simulink model "PIME_FxNLMS_2023a"  (R2023a)
settings: Solver=VariableStepAuto  StartTime=0.0  StopTime=60  FixedStep=1/fs  RelTol=1e-3
values from neighbouring files (symbols this model uses):
  alpha = 0.999    [pime_init.m]
  c2 = 0.12    [pime_init.m]
  fs = 2000    [pime_init.m]
  k = 0.06    [pime_init.m]
  Mp = 500    [pime_init.m]
  Ms = 500    [pime_init.m]
  mu = 0.4    [pime_init.m]
  mu2 = 0.1    [pime_init.m]
  pp_mic4 = [-0.00152613187005 0.000492531757844 -0.000591319109315 0.000123902983694 0.000500734431321 -0.00102276849056 0.00131789801081 -0.000708342152862 0.00106442677388 -0.0010811148944 0.00122345086739 -0.00108254398921 ... (2000 elements, 2000x1)]    [paths_2kHz_mic643.mat]
  pp_mic6 = [0.00546659867813 -0.00630560555543 0.00626955740335 -0.00617656797871 0.00600172736047 -0.00577131330306 0.00631697277776 -0.0055608004128 0.00521354039728 -0.00486275779688 0.00518931562889 -0.00454952673028 ... (2000 elements, 2000x1)]    [paths_2kHz_mic643.mat]
  sp_mic4 = [0.0248657891061 -0.0218126639931 0.0255846134288 -0.0178527223693 0.0231404239645 0.863574751981 -0.0887369954303 -0.473837577644 -0.356836562663 -0.384364342858 -0.167933167392 -0.0752079364537 ... (2000 elements, 2000x1)]    [paths_2kHz_mic643.mat]
  sp_mic6 = [0.0393906263967 -0.0418257652999 0.0388004904193 -0.0450848758925 0.464349566334 1.5072784377 -0.746160308217 -0.827489248229 -0.750534401853 -0.550302899738 -0.217506295103 -0.0688944606907 ... (2000 elements, 2000x1)]    [paths_2kHz_mic643.mat]
  t_mic_change = 30    [pime_init.m]
undefined symbols (not defined in the file or in its folder): pp_micro6, sp_micro6
libraries: simulink x3, dspadpt3 x2, dspswit3 x2, dspsrcs4 x1, dspvision x1
settings Model: Creator=JUAGA26J  LastModifiedBy=enrole
settings DataIOCC: SaveFormat=Array
settings RTWCC: GPUComputeCapability=5.0

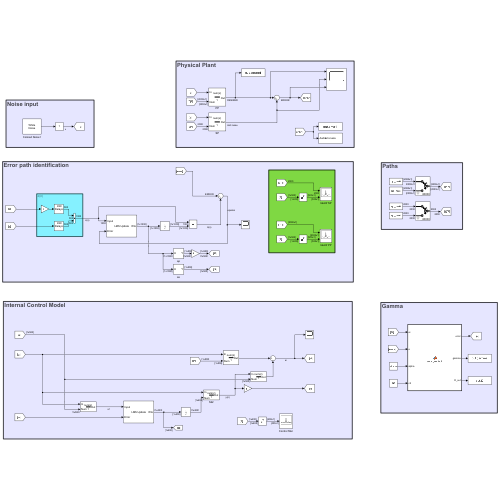
[thumbnail: Simulink's stored preview of the top-level diagram]
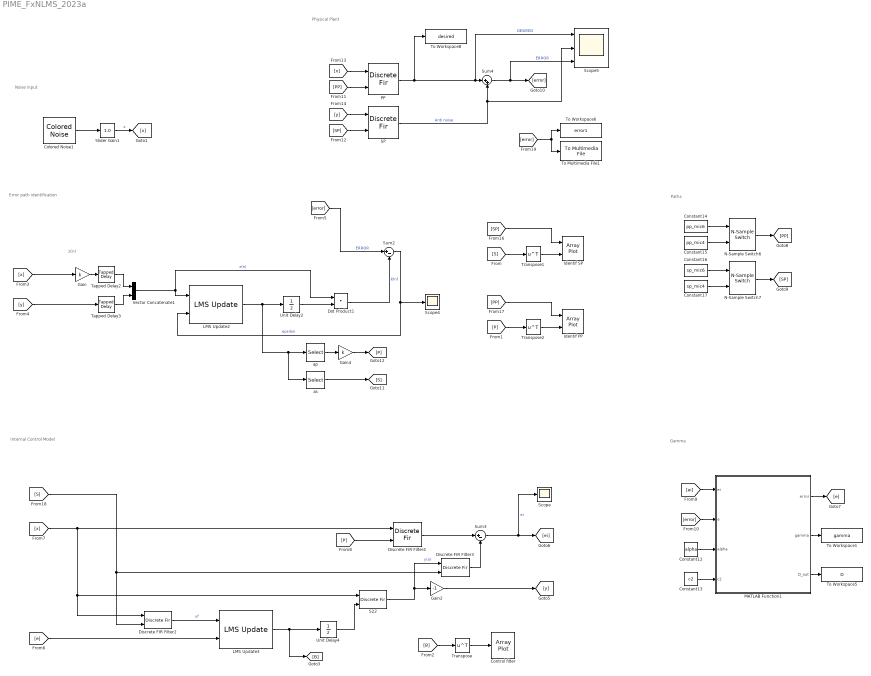
== system PIME_FxNLMS_2023a ==
  note: Physical Plant
  note: Paths
  note: Gamma
  note: Internal Control Model
  note: Noise input
  note: Error path identification
  note: z(n)
  Colored Noise1 : dspsrcs4/Colored Noise  Color=white  InverseFrequencyPower=1  BoundedOutput=on  NumChannels=1  OutputDataType=double  SamplesPerFrame=1  SampleTime=1/fs  RandomStream=mt19937ar with seed  Seed=877  SimulateUsing=Code generation
      settings: LibrarySourceBlock=audiosources/Colored Noise
  Constant12 : Constant  Value=alpha
  Constant13 : Constant  Value=c2
  Constant14 : Constant  Value=pp_mic6  VectorParams1D=off  SampleTime=1/fs
  Constant15 : Constant  Value=pp_mic4  VectorParams1D=off  SampleTime=1/fs
  Constant16 : Constant  Value=sp_mic6  SampleTime=1/fs
  Constant17 : Constant  Value=sp_mic4  SampleTime=1/fs
  Control filter : ArrayPlot  WindowPosition=[1.000000,41.000000,1920.000000,1017.000000,]  ScopeFrameLocation=window  YLimits=[-0.0937,0.0836]  ShowLegend=on
      settings: OpenAtSimulationStart=off
  Discrete FIR Filter2 : DiscreteFir  CoefSource=Input port
      settings: InputPortMap=u0,u1
  Discrete FIR Filter3 : DiscreteFir  CoefSource=Input port
      settings: InputPortMap=u0,u1
  Discrete FIR Filter4 : DiscreteFir  CoefSource=Input port
      settings: InputPortMap=u0,u1
  Dot Product1 : DotProduct  OutDataTypeStr=Inherit: Inherit via internal rule
  Gain : Gain  Gain=k
  Gain2 : Gain  Gain=-1
  Gain4 : Gain  Gain=k
  Identif PP : ArrayPlot  NumInputPorts=2  WindowPosition=[1.000000,49.000000,1920.000000,1009.000000,]  ScopeFrameLocation=window  MaximizeAxes=Off  YLimits=[-0.0933,0.0799]  ShowLegend=on
      settings: OpenAtSimulationStart=off
  Identif SP : ArrayPlot  NumInputPorts=2  WindowPosition=[1.000000,49.000000,1920.000000,1009.000000,]  ScopeFrameLocation=window  YLimits=[-0.8419,1.2914]  ShowLegend=on
      settings: OpenAtSimulationStart=off
  LMS Update2 : dspadpt3/LMS Update  Method=Normalized LMS  Length=L  NumFilters=1  StepSizeSource=Property  StepSize=mu  LeakageFactor=1  InitialConditions=Initial  AdaptiveFilterMode=Adaptive linear combiner  EnableAdaptInput=off  EnableResetInput=off  SimulateUsing=Interpreted execution
  LMS Update3 : dspadpt3/LMS Update  Method=Normalized LMS  Length=L2  NumFilters=1  StepSizeSource=Property  StepSize=mu2  LeakageFactor=1  InitialConditions=0  AdaptiveFilterMode=Tapped delay-line FIR filter  EnableAdaptInput=off  EnableResetInput=off  SimulateUsing=Interpreted execution
  MATLAB Function1 : MATLAB Function  TreatAsAtomicUnit=on
  N-Sample Switch6 : dspswit3/N-Sample Switch  N=t_mic_change*fs  reset=off  TriggerType=Rising edge  Ts=1/fs
  N-Sample Switch7 : dspswit3/N-Sample Switch  N=t_mic_change*fs  reset=off  TriggerType=Rising edge  Ts=1/fs
  PP : DiscreteFir  CoefSource=Input port  Coefficients=pp_micro6
      settings: InputPortMap=u0,u1
  S22 : DiscreteFir  CoefSource=Input port
      settings: InputPortMap=u0,u1
  SP : DiscreteFir  CoefSource=Input port  Coefficients=sp_micro6
      settings: InputPortMap=u0,u1
  Scope : Scope
  Scope4 : Scope
  Scope5 : Scope  NumInputPorts=3
  Slider Gain1 : simulink/Math Operations/Slider Gain  gain=1.0  low=0  high=10
  Sum2 : Sum  Inputs=|+-
  Sum3 : Sum  Inputs=|+-
  Sum4 : Sum  Inputs=|++
  Tapped Delay2 : simulink/Discrete/Tapped Delay  vinit=0  samptime=-1  NumDelays=Mp-1  DelayOrder=Newest  includeCurrent=on
  Tapped Delay3 : simulink/Discrete/Tapped Delay  vinit=0  samptime=-1  NumDelays=Ms-1  DelayOrder=Newest  includeCurrent=on
  To Multimedia File1 : dspvision/To Multimedia File  outputFilename=error.wav  streamSelection=Audio only  videoCompressor=None (uncompressed)  audioCompressor=None (uncompressed)  imagePorts=Separate color signals  fileType=WAV  audioDatatype=16-bit integer  fourcc=RGB  videoQuality=75  mj2000CompFactor=10
      settings: LibrarySourceBlock=audiosinks/To Multimedia File
  To Workspace1 : ToWorkspace  VariableName=gamma  SampleTime=-1
      settings: Save2DSignal=2-D array (concatenate along first dimension)
  To Workspace5 : ToWorkspace  VariableName=D  SampleTime=-1
      settings: Save2DSignal=2-D array (concatenate along first dimension)
  To Workspace6 : ToWorkspace  VariableName=error1  SampleTime=-1
      settings: Save2DSignal=2-D array (concatenate along first dimension)
  To Workspace8 : ToWorkspace  VariableName=desired  SampleTime=-1
      settings: Save2DSignal=2-D array (concatenate along first dimension)
  Transpose : Math  Operator=transpose
  Transpose1 : Math  Operator=transpose
  Transpose2 : Math  Operator=transpose
  Unit Delay2 : UnitDelay  SampleTime=-1
  Unit Delay4 : UnitDelay  SampleTime=-1
  Vector Concatenate1 : Concatenate
  ap : Selector  InputPortWidth=1000  IndexOptions=Index vector (dialog)  Indices=[1:500]  OutputSizes=1
  as : Selector  InputPortWidth=1000  IndexOptions=Index vector (dialog)  Indices=[501:1000]  OutputSizes=1
  wires:
  [S] -> Transpose1/1
  [SP] -> Identif SP/1
  Transpose1/1 -> Identif SP/2
  [PP] -> Identif PP/1
  Transpose2/1 -> Identif PP/2
  [P] -> Transpose2/1
  [B] -> Transpose/1
  Transpose/1 -> Control filter/1
  Vector Concatenate1/1 -> LMS Update2/1, Dot Product1/1  "z(n)"
  LMS Update2/1 -> as/1, ap/1, Unit Delay2/1
  Dot Product1/1 -> Sum2/2  "ê(n)"
  Unit Delay2/1 -> Dot Product1/2
  [error] -> Sum2/1  "ERROR"
  Sum2/1 -> LMS Update2/2, Scope4/1  "epsilon"
  Tapped Delay2/1 -> Vector Concatenate1/1
  [y] -> Tapped Delay3/1
  Tapped Delay3/1 -> Vector Concatenate1/2
  [x] -> Gain/1
  Gain/1 -> Tapped Delay2/1
  Colored Noise1/1 -> Slider Gain1/1
  Slider Gain1/1 -> [x]  "x"
  Discrete FIR Filter3/1 -> Sum3/2
  Discrete FIR Filter4/1 -> Sum3/1
  Unit Delay4/1 -> S22/2
  S22/1 -> Gain2/1, Discrete FIR Filter3/1  "y(n)"
  [S] -> Discrete FIR Filter3/2, Discrete FIR Filter2/2
  LMS Update3/1 -> Unit Delay4/1, [B]
  Sum3/1 -> Scope/1, [ei]  "ei"
  Discrete FIR Filter2/1 -> LMS Update3/1  "xf"
  [x] -> Discrete FIR Filter2/1, S22/1, Discrete FIR Filter4/1
  [e] -> LMS Update3/2
  Gain2/1 -> [y]
  [ei] -> MATLAB Function1/1(ei)
  Constant13/1 -> MATLAB Function1/4(c2)
  Constant12/1 -> MATLAB Function1/3(alpha)
  MATLAB Function1/1(error) -> [e]
  [error] -> MATLAB Function1/2(e)
  Constant14/1 -> N-Sample Switch6/1
  N-Sample Switch6/1 -> [PP]
  Constant15/1 -> N-Sample Switch6/2
  N-Sample Switch7/1 -> [SP]
  Constant16/1 -> N-Sample Switch7/1
  Constant17/1 -> N-Sample Switch7/2
  [P] -> Discrete FIR Filter4/2
  [SP] -> SP/2
  [PP] -> PP/2
  [x] -> PP/1
  [y] -> SP/1
  PP/1 -> Scope5/1, Sum4/1, To Workspace8/1  "DESIRED"
  SP/1 -> Scope5/2, Sum4/2  "Anti noise"
  Sum4/1 -> [error], Scope5/3  "ERROR"
  as/1 -> [S]
  ap/1 -> Gain4/1
  Gain4/1 -> [P]
  MATLAB Function1/2(gamma) -> To Workspace1/1
  MATLAB Function1/3(D_out) -> To Workspace5/1
  [error] -> To Workspace6/1, To Multimedia File1/1

== matlab function PIME_FxNLMS_2023a/MATLAB Function1 ==
  data: ei input; error output; e input; gamma output; D_out output; alpha input; c2 input

function [error, gamma, D_out] = error_control(ei, e, alpha, c2)

persistent D

if isempty (D)
    D=0;
end

D=max(abs(ei),alpha*D+(1-alpha)*abs(ei));
gamma=1-(D/(D+c2));
% gamma=0;
error=gamma*e+(1-gamma)*ei;
D_out=D;
